simulink model "rlc"  (R2025a)
settings: Solver=ode23  StartTime=0.0  StopTime=0.2  RelTol=1e-3
libraries: spsSeriesRLCBranchLib x30, spsCurrentMeasurementLib x8, spsDCVoltageSourceLib x8, spsVoltageMeasurementLib x8, spsControlledCurrentSourceLib x4, sps_lib x1
settings Model: Creator=simlab2025  LastModifiedBy=aayus
settings SolverCC: AlgebraicLoopSolver=TrustRegion
settings DataIOCC: ReturnWorkspaceOutputs=off
settings DebuggingCC: UnconnectedInputMsg=warning  UnconnectedOutputMsg=warning  UnconnectedLineMsg=warning  ArithmeticOperatorsInVariantConditions=warning
settings ModelReferenceCC: EnableRefExpFcnMdlSchedulingChecks=on
settings SFSimCC: SimUseLocalCustomCode=off  CustomCodeUndefinedFunction=UseInterfaceOnly
settings RTWCC: RTWUseLocalCustomCode=off  GPUComputeCapability=3.5

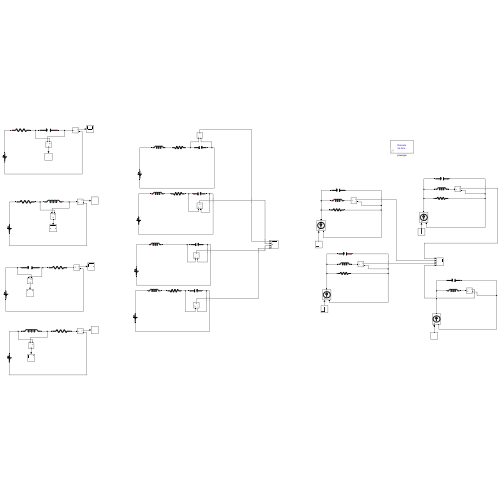
[thumbnail: Simulink's stored preview of the top-level diagram]
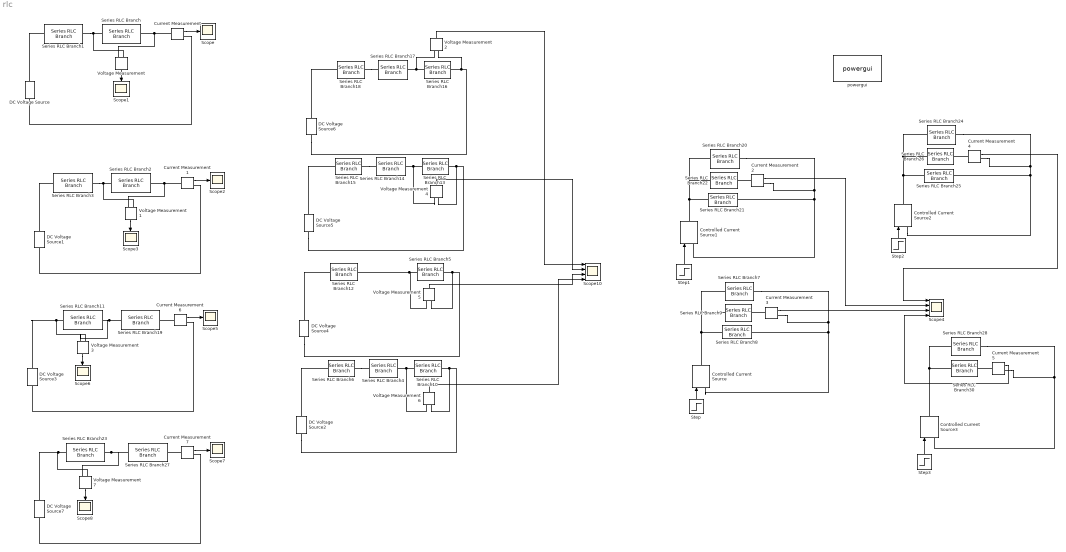
== system rlc ==
  Controlled Current Source{,1..3} (4 alike) : spsControlledCurrentSourceLib/Controlled Current Source  Initialize=on  Source_Type=AC  Amplitude=0  Phase=0  Frequency=0  Measurements=None
  Current Measurement{,1..7} (8 alike) : spsCurrentMeasurementLib/Current Measurement  PhasorSimulation=off  OutputType=Complex  PSBequivalent=0
  DC Voltage Source{,1..7} (8 alike) : spsDCVoltageSourceLib/DC Voltage Source  Amplitude=10  Measurements=None
  Scope{,1..3,5..8} (8 alike) : Scope
      Scope settings: ActiveDisplayYMinimum=-0.00012499999753630935  ActiveDisplayYMaximum=0.0011249999997262566
      Scope1 settings: ActiveDisplayYMinimum=-10.91387  ActiveDisplayYMaximum=0.60088
      Scope2 settings: ActiveDisplayYMinimum=-0.01249999997423178  ActiveDisplayYMaximum=0.11249999976808606  DataLoggingVariableName=ScopeData2
      Scope3 settings: ActiveDisplayYMinimum=-10.91387  ActiveDisplayYMaximum=0.60088  DataLoggingVariableName=ScopeData3
      Scope5 settings: ActiveDisplayYMinimum=-0.00012499999768092706  ActiveDisplayYMaximum=0.0011249999997423254  DataLoggingVariableName=ScopeData5
      Scope6 settings: ActiveDisplayYMinimum=-10.91387  ActiveDisplayYMaximum=0.60088  DataLoggingVariableName=ScopeData6
      Scope7 settings: ActiveDisplayYMinimum=-0.01249999997423178  ActiveDisplayYMaximum=0.11249999976808606  DataLoggingVariableName=ScopeData7
      Scope8 settings: ActiveDisplayYMinimum=-10.91387  ActiveDisplayYMaximum=0.60088  DataLoggingVariableName=ScopeData8
  Scope10 : Scope  NumInputPorts=4
      settings: ActiveDisplayYMinimum=-2.49996  ActiveDisplayYMaximum=22.49996  DataLoggingVariableName=ScopeData10
  Scope4 : Scope  NumInputPorts=4
      settings: ActiveDisplayYMinimum=-2.5  ActiveDisplayYMaximum=22.49996  DataLoggingVariableName=ScopeData4
  Series RLC Branch : spsSeriesRLCBranchLib/Series RLC Branch  LConnTagsString=__new0  RConnTagsString=__new0  BranchType=C  Resistance=1  Inductance=1e-3  SetiL0=on  InitialCurrent=0  Capacitance=1e-6  Setx0=on  InitialVoltage=0  Measurements=None
  Series RLC Branch1 : spsSeriesRLCBranchLib/Series RLC Branch  LConnTagsString=__new0  RConnTagsString=__new0  BranchType=R  Resistance=10000  Inductance=0  SetiL0=off  InitialCurrent=0  Capacitance=0  Setx0=off  InitialVoltage=0  Measurements=None
  Series RLC Branch{5,10,13,16} (4 alike) : spsSeriesRLCBranchLib/Series RLC Branch  LConnTagsString=__new0  RConnTagsString=__new0  BranchType=C  Resistance=20  Inductance=1  SetiL0=on  InitialCurrent=0  Capacitance=1e-6  Setx0=on  InitialVoltage=0  Measurements=None
  Series RLC Branch11 : spsSeriesRLCBranchLib/Series RLC Branch  LConnTagsString=__new0  RConnTagsString=__new0  BranchType=C  Resistance=1  Inductance=1e-3  SetiL0=on  InitialCurrent=0  Capacitance=1e-6  Setx0=on  InitialVoltage=0  Measurements=None
  Series RLC Branch{6,9,12,15,18,22,26,30} (8 alike) : spsSeriesRLCBranchLib/Series RLC Branch  LConnTagsString=__new0  RConnTagsString=__new0  BranchType=L  Resistance=200  Inductance=1  SetiL0=on  InitialCurrent=0  Capacitance=0  Setx0=off  InitialVoltage=0  Measurements=None
  Series RLC Branch14 : spsSeriesRLCBranchLib/Series RLC Branch  LConnTagsString=__new0  RConnTagsString=__new0  BranchType=R  Resistance=20  Inductance=1  SetiL0=on  InitialCurrent=0  Capacitance=1e-6  Setx0=on  InitialVoltage=0  Measurements=None
  Series RLC Branch17 : spsSeriesRLCBranchLib/Series RLC Branch  LConnTagsString=__new0  RConnTagsString=__new0  BranchType=R  Resistance=2000  Inductance=1  SetiL0=on  InitialCurrent=0  Capacitance=1e-6  Setx0=on  InitialVoltage=0  Measurements=None
  Series RLC Branch19 : spsSeriesRLCBranchLib/Series RLC Branch  LConnTagsString=__new0  RConnTagsString=__new0  BranchType=R  Resistance=10000  Inductance=0  SetiL0=off  InitialCurrent=0  Capacitance=0  Setx0=off  InitialVoltage=0  Measurements=None
  Series RLC Branch2 : spsSeriesRLCBranchLib/Series RLC Branch  LConnTagsString=__new0  RConnTagsString=__new0  BranchType=L  Resistance=1  Inductance=1  SetiL0=on  InitialCurrent=0  Capacitance=1e-6  Setx0=on  InitialVoltage=0  Measurements=None
  Series RLC Branch{7,20,24,28} (4 alike) : spsSeriesRLCBranchLib/Series RLC Branch  LConnTagsString=__new0  RConnTagsString=__new0  BranchType=C  Resistance=5  Inductance=1  SetiL0=on  InitialCurrent=0  Capacitance=1e-6  Setx0=on  InitialVoltage=0  Measurements=None
  Series RLC Branch21 : spsSeriesRLCBranchLib/Series RLC Branch  LConnTagsString=__new0  RConnTagsString=__new0  BranchType=R  Resistance=20  Inductance=1  SetiL0=on  InitialCurrent=0  Capacitance=0  Setx0=off  InitialVoltage=0  Measurements=None
  Series RLC Branch23 : spsSeriesRLCBranchLib/Series RLC Branch  LConnTagsString=__new0  RConnTagsString=__new0  BranchType=L  Resistance=1  Inductance=1  SetiL0=on  InitialCurrent=0  Capacitance=1e-6  Setx0=on  InitialVoltage=0  Measurements=None
  Series RLC Branch25 : spsSeriesRLCBranchLib/Series RLC Branch  LConnTagsString=__new0  RConnTagsString=__new0  BranchType=R  Resistance=200  Inductance=1  SetiL0=on  InitialCurrent=0  Capacitance=0  Setx0=off  InitialVoltage=0  Measurements=None
  Series RLC Branch27 : spsSeriesRLCBranchLib/Series RLC Branch  LConnTagsString=__new0  RConnTagsString=__new0  BranchType=R  Resistance=100  Inductance=0  SetiL0=off  InitialCurrent=0  Capacitance=0  Setx0=off  InitialVoltage=0  Measurements=None
  Series RLC Branch3 : spsSeriesRLCBranchLib/Series RLC Branch  LConnTagsString=__new0  RConnTagsString=__new0  BranchType=R  Resistance=100  Inductance=0  SetiL0=off  InitialCurrent=0  Capacitance=0  Setx0=off  InitialVoltage=0  Measurements=None
  Series RLC Branch4 : spsSeriesRLCBranchLib/Series RLC Branch  LConnTagsString=__new0  RConnTagsString=__new0  BranchType=R  Resistance=200000  Inductance=1  SetiL0=on  InitialCurrent=0  Capacitance=1e-6  Setx0=on  InitialVoltage=0  Measurements=None
  Series RLC Branch8 : spsSeriesRLCBranchLib/Series RLC Branch  LConnTagsString=__new0  RConnTagsString=__new0  BranchType=R  Resistance=20000  Inductance=1  SetiL0=on  InitialCurrent=0  Capacitance=0  Setx0=off  InitialVoltage=0  Measurements=None
  Step : Step  Time=0.01  After=10  SampleTime=0
  Step1 : Step  Time=0.01  After=10  SampleTime=0
  Step2 : Step  Time=0  After=10  SampleTime=0.2
  Step3 : Step  Time=0.01  After=10  SampleTime=0
  Voltage Measurement{,1..7} (8 alike) : spsVoltageMeasurementLib/Voltage Measurement  PhasorSimulation=off  OutputType=Complex  PSBequivalent=0
  powergui : sps_lib/powergui  Priority=1  SimulationMode=Discrete  SampleTime=50e-7  frequency=50  Iterations=50  frequencyindice=0  Pbase=100e6  ErrMax=1e-4  UnitsV=kV  UnitsW=MW  buscounter=0  FunctionMessages=off  echomessages=off  EnableUseOfTLC=off  CurrentSourceSwitches=off  DisableSnubberDevices=off  DisableRonSwitches=off  DisableVfSwitches=off  DisplayEquations=off  AutomaticDiscreteSolvers=off  SolverType=Tustin/Backward Euler (TBE)  Interpol=off  ExternalGateDelay=off  methode=off  Ts=100  x0status=blocks  SPID=on  SwTol=0  HookPort=off  NonlinearTolerance=1e-4  nMaxIteration=100  ContinueOnMaxIteration=off  RestoreLinks=warning  ResistiveCurrentMeasurement=off  Frange=[0:2:500]  Ylog=off  Xlog=on  ShowGrid=off  save=off  variable=ZData  structure=0  ZoomFFT=off  StartTime=0.0  cycles=1  DisplayStyle=1  fundamental=60  FreqAxis=off  MaxFrequency=1000  frequencyindicesteady=1  RmsSteady=1  display=off
  wires:
  Current Measurement/1 -> Scope/1
  Voltage Measurement/1 -> Scope1/1
  Current Measurement1/1 -> Scope2/1
  Voltage Measurement1/1 -> Scope3/1
  Voltage Measurement6/1 -> Scope10/4
  Voltage Measurement5/1 -> Scope10/3
  Voltage Measurement4/1 -> Scope10/2
  Voltage Measurement2/1 -> Scope10/1
  Step/1 -> Controlled Current Source/1
  Current Measurement4/1 -> Scope4/1
  Current Measurement5/1 -> Scope4/4
  Current Measurement2/1 -> Scope4/2
  Current Measurement3/1 -> Scope4/3
  Step1/1 -> Controlled Current Source1/1
  Step3/1 -> Controlled Current Source3/1
  Step2/1 -> Controlled Current Source2/1
  Voltage Measurement3/1 -> Scope6/1
  Current Measurement6/1 -> Scope5/1
  Current Measurement7/1 -> Scope7/1
  Voltage Measurement7/1 -> Scope8/1
  connections:
  Current Measurement/LConn1 -- Voltage Measurement/LConn2 -- Series RLC Branch/LConn1
  Current Measurement/RConn1 -- DC Voltage Source/LConn1
  Series RLC Branch1/LConn1 -- DC Voltage Source/RConn1
  Voltage Measurement/LConn1 -- Series RLC Branch1/RConn1 -- Series RLC Branch/RConn1
  Current Measurement1/LConn1 -- Voltage Measurement1/LConn2 -- Series RLC Branch2/LConn1
  Voltage Measurement1/LConn1 -- Series RLC Branch3/RConn1 -- Series RLC Branch2/RConn1
  Current Measurement1/RConn1 -- DC Voltage Source1/LConn1
  Series RLC Branch3/LConn1 -- DC Voltage Source1/RConn1
  Series RLC Branch10/LConn1 -- Voltage Measurement6/LConn1 -- Series RLC Branch4/LConn1
  Series RLC Branch6/RConn1 -- Series RLC Branch4/RConn1
  DC Voltage Source2/RConn1 -- Series RLC Branch6/LConn1
  DC Voltage Source2/LConn1 -- Voltage Measurement6/LConn2 -- Series RLC Branch10/RConn1
  Series RLC Branch5/LConn1 -- Series RLC Branch12/RConn1 -- Voltage Measurement5/LConn1
  DC Voltage Source4/RConn1 -- Series RLC Branch12/LConn1
  DC Voltage Source4/LConn1 -- Voltage Measurement5/LConn2 -- Series RLC Branch5/RConn1
  Series RLC Branch15/RConn1 -- Series RLC Branch14/RConn1
  DC Voltage Source5/RConn1 -- Series RLC Branch15/LConn1
  DC Voltage Source5/LConn1 -- Voltage Measurement4/LConn2 -- Series RLC Branch13/RConn1
  Series RLC Branch13/LConn1 -- Voltage Measurement4/LConn1 -- Series RLC Branch14/LConn1
  Series RLC Branch18/RConn1 -- Series RLC Branch17/RConn1
  DC Voltage Source6/RConn1 -- Series RLC Branch18/LConn1
  DC Voltage Source6/LConn1 -- Voltage Measurement2/LConn2 -- Series RLC Branch16/RConn1
  Series RLC Branch16/LConn1 -- Voltage Measurement2/LConn1 -- Series RLC Branch17/LConn1
  Series RLC Branch8/LConn1 -- Controlled Current Source/RConn1 -- Series RLC Branch7/RConn1 -- Series RLC Branch9/LConn1
  Series RLC Branch7/LConn1 -- Controlled Current Source/LConn1 -- Series RLC Branch8/RConn1 -- Current Measurement3/RConn1
  Current Measurement3/LConn1 -- Series RLC Branch9/RConn1
  Series RLC Branch21/LConn1 -- Controlled Current Source1/RConn1 -- Series RLC Branch20/RConn1 -- Series RLC Branch22/LConn1
  Current Measurement2/LConn1 -- Series RLC Branch22/RConn1
  Series RLC Branch24/LConn1 -- Current Measurement4/RConn1 -- Controlled Current Source2/LConn1 -- Series RLC Branch25/RConn1
  Series RLC Branch25/LConn1 -- Controlled Current Source2/RConn1 -- Series RLC Branch24/RConn1 -- Series RLC Branch26/LConn1
  Current Measurement4/LConn1 -- Series RLC Branch26/RConn1
  Series RLC Branch28/LConn1 -- Current Measurement5/RConn1 -- Controlled Current Source3/LConn1
  Series RLC Branch30/LConn1 -- Controlled Current Source3/RConn1 -- Series RLC Branch28/RConn1
  Current Measurement5/LConn1 -- Series RLC Branch30/RConn1
  Series RLC Branch20/LConn1 -- Current Measurement2/RConn1 -- Controlled Current Source1/LConn1 -- Series RLC Branch21/RConn1
  Series RLC Branch11/LConn1 -- Series RLC Branch19/LConn1 -- Voltage Measurement3/LConn2
  Series RLC Branch11/RConn1 -- Voltage Measurement3/LConn1 -- DC Voltage Source3/RConn1
  Current Measurement6/RConn1 -- DC Voltage Source3/LConn1
  Current Measurement6/LConn1 -- Series RLC Branch19/RConn1
  Series RLC Branch23/RConn1 -- DC Voltage Source7/RConn1 -- Voltage Measurement7/LConn1
  Series RLC Branch23/LConn1 -- Series RLC Branch27/LConn1 -- Voltage Measurement7/LConn2
  Current Measurement7/RConn1 -- DC Voltage Source7/LConn1
  Current Measurement7/LConn1 -- Series RLC Branch27/RConn1
